simulink model "FCSMPC_double_vector_2025b"  (R2025b)
settings: Solver=FixedStepDiscrete  StartTime=0.0  StopTime=2  FixedStep=SimulinkTs  RelTol=1e-3
PreLoadFcn:
  | % Verzeichnis des Modells zum MATLAB-Pfad hinzufügen
  | modelDir = fileparts(get_param(bdroot, 'FileName'));
  | addpath(modelDir);
  | 
  | % Nur der Dateiname – kein Pfad!
  | set_param(bdroot, 'DataDictionary', 'FOC_params.sldd');
model workspace (MAT data in the model file):
  Np : Simulink.Parameter (value not decoded)
values from neighbouring files (symbols this model uses):
  Filter_Current_FilterTimeConst = 3.3333333333333335E-5    [FOC_params.sldd]
  Filter_Current_SensorTimeConst = 1.5915494309189535E-6    [FOC_params.sldd]
  FOC = evalin("base", "FOC")    [createFOC_SLDD.m]
  FOC_Control_Current_KIid = 10.0    [FOC_params.sldd]
  FOC_Control_Current_KIiq = 10.0    [FOC_params.sldd]
  FOC_Control_Current_KPid = 0.20418507462686566    [FOC_params.sldd]
  FOC_Control_Current_KPiq = 0.58674626865671642    [FOC_params.sldd]
  FOC_Control_Current_Krd = 0.8    [FOC_params.sldd]
  FOC_Control_Current_Krq = 0.8    [FOC_params.sldd]
  FOC_Control_Current_TclCur = 0.1    [FOC_params.sldd]
  FOC_Control_Current_Tnd = 0.1    [FOC_params.sldd]
  FOC_Control_Current_Tnq = 0.1    [FOC_params.sldd]
  FOC_Control_InverterVdc_V = 400.0    [FOC_params.sldd]
  FOC_Control_MotorImax_A = 650.0    [FOC_params.sldd]
  FOC_Control_MTPA_MTPV_nT_id_grid = -450.06704889786266 -439.56177000270145 -427.77784873303676 -416.66404703197372 -406.07553272717422 -395.15516533678584 -384.31176061747851 -374.03652088128132 -363.90551910193739 -353.79478643334204 -344.0221683092833 -334.51243453441936 -324.94614350292119 -315.21793409137081 -305.26543360965195 -295.21828280911944 -285.133916324101 -275.01232812136521 -264.86951532374729 -254.7797625148454 -244    [FOC_params.sldd]
  FOC_Control_MTPA_MTPV_nT_iq_grid = -449.09165648258488 -442.56958748923387 -437.25247759546528 -430.91792082419158 -423.83735797306491 -417.11730433547 -410.54064621830616 -403.71584331167304 -396.93611069310379 -390.15794305727007 -382.97216593027133 -375.44639668848538 -367.93447385667577 -360.57088856352266 -353.41289778449368 -346.34020584402072 -339.28416684923008 -332.22010880540631 -325.11927997033376 -317.92299905654966 -31    [FOC_params.sldd]
  FOC_Control_MTPA_MTPV_T_vec = -245.0 -240.0 -235.0 -230.0 -225.0 -220.0 -215.0 -210.0 -205.0 -200.0 -195.0 -190.0 -185.0 -180.0 -175.0 -170.0 -165.0 -160.0 -155.0 -150.0 -145.0 -140.0 -135.0 -130.0 -125.0 -120.0 -115.0 -110.0 -105.0 -100.0 -95.0 -90.0 -85.0 -80.0 -75.0 -70.0 -65.0 -60.0 -55.0 -50.0 -45.0 -40.0 -35.0 -30.0 -25.0 -20.0 -15.0 -10.0 -5.0 0.0 5.0 10.0 15.0 20.0 25.0 30.0 35.0 40.0 45.0 50.0 55.0 60.0 65.0 70.0 75.0    [FOC_params.sldd]
  FOC_Control_MTPA_MTPV_w_vec = 0.0 10.471975511965978 20.943951023931955 31.415926535897931 41.887902047863911 52.359877559829883 62.831853071795862 73.303828583761828 83.775804095727821 94.247779607693786 104.71975511965977 115.19173063162575 125.66370614359172 136.1356816555577 146.60765716752366 157.07963267948966 167.55160819145564 178.02358370342159 188.49555921538757 198.96753472735358 209.43951023931953 219.9114857512855    [FOC_params.sldd]
  FOC_Control_OpenLoop_Id_Ref_A = 0.0    [FOC_params.sldd]
  FOC_Control_OpenLoop_Iq_Ref_A = 0.0    [FOC_params.sldd]
  FOC_Control_OpenLoop_Ud_OpenLoop_V = 0.0    [FOC_params.sldd]
  FOC_Control_OpenLoop_Uq_OpenLoop_V = 0.0    [FOC_params.sldd]
  FOC_Control_RF_omegamech_rad_s = 3141.5926535897934    [FOC_params.sldd]
  FOC_Control_RF_RateCurrent_A = 500.0    [FOC_params.sldd]
  FOC_Control_RF_RateTrq_Nm = 500.0    [FOC_params.sldd]
  FOC_Control_theta_mechOffsetFix = 0.0    [FOC_params.sldd]
  FOC_Control_theta_mechOffsetTime = 0.0    [FOC_params.sldd]
  FOC_Control_TorqueRef_Nm = 10.0    [FOC_params.sldd]
  FOC_Control_Umax_V = 230.94010767585033    [FOC_params.sldd]
  FOC_Flag_ClosedLoopControl = 1.0    [FOC_params.sldd]
  FOC_Flag_ControlStrategy = 2.0    [FOC_params.sldd]
  FOC_Flag_PWMEnable = 1.0    [FOC_params.sldd]
  FOC_Flag_ResetControl = 0.0    [FOC_params.sldd]
  FOC_Flag_TorqueControl = 1.0    [FOC_params.sldd]
  FOC_LUT_DQLimiter_DQ_LUTScaling = 1.8749999999999995E-5    [FOC_params.sldd]
  FOC_PWM_AZSPWMMethod = 3.0    [FOC_params.sldd]
  FOC_PWM_HybridMode = 1.0    [FOC_params.sldd]
  FOC_PWM_LB1 = 0.5    [FOC_params.sldd]
  FOC_PWM_LB2 = 0.77    [FOC_params.sldd]
  FOC_PWM_PWMManuel = 1.0    [FOC_params.sldd]
  FOC_PWM_RSPWMMethod = 2.0    [FOC_params.sldd]
  FOC_PWM_UB1 = 0.66    [FOC_params.sldd]
  FOC_PWM_UB2 = 0.9    [FOC_params.sldd]
  FOC_SampleTime_TsCur = 0.0001    [FOC_params.sldd]
undefined symbols (not defined in the file or in its folder): dspblkCoreblockFVToolHelper, FCS, Filter, gcbh, Plant, SimulinkTs
libraries: hdlsllib x2, simulink x2, autolibfluxpmsm x1
(part 5 of 8)

== matlab function FCSMPC_double_vector_2025b/FCS_MPC/SDA_Solve/SDA Solve/QP_Runtime_40k_Simplified ==
  data: H input double size=[15 15]; U_unc output double size=[15 1]; Gamma input double size=[10 2]; Phi input double size=[10 1]; Lambdafsw_SE input double size=[15 3]; Upsil input double size=[10 15]; Bd input double size=[2 2]; Bs_TI input double size=[2 3]; deltaIdqBaseOffset input double size=[2 1]; deltaIdqState input double size=[2 2]; magnitudeGain input double size=[1 1]; phaseCompensation input double size=[2 2]; rippleAttenuation input double size=[1 1]; rippleDelay input double size=[1 1]; Sin_Cos_Theta input double size=[2 1]; idiqFiltered input double size=[2 1]; idiq_ref input double size=[2 1]; Ts input double size=[1 1]; U_applied input double size=[6 1]; controllerDelay input double size=[1 1]; iabcPredictedPrevious input double size=[3 1]; Iabc_Motor input double size=[3 1]; predictionValid input boolean size=[1 1]; iabcReconstruction output double size=[3 1]; deltaIabcBase output double size=[3 1]; deltaIabcSwitch output double size=[3 3]; predictionError output double size=[3 1]; reconstructionError output double size=[3 1]; predictionError_dq output double size=[2 1]; reconstructionError_dq output double size=[2 1]; iabcAverageEstimated output double size=[3 1]; iabcRippleEstimated output double size=[3 1]; rippleResidual output double size=[3 1]; iabcSwitchCorrectionRaw output double size=[3 1]
function [U_unc,iabcReconstruction, ...
    deltaIabcBase,deltaIabcSwitch, ...
    predictionError,reconstructionError, ...
    predictionError_dq,reconstructionError_dq, ...
    iabcAverageEstimated,iabcRippleEstimated,rippleResidual, ...
    iabcSwitchCorrectionRaw] = ...
    QP_Runtime_40k_Simplified( ...
    H,Gamma,Phi,Lambdafsw_SE,Upsil,Bd,Bs_TI, ...
    deltaIdqBaseOffset,deltaIdqState, ...
    magnitudeGain,phaseCompensation,rippleAttenuation,rippleDelay, ...
    Sin_Cos_Theta,idiqFiltered,idiq_ref,Ts,U_applied,controllerDelay, ...
    iabcPredictedPrevious,Iabc_Motor,predictionValid)
%#codegen
% Fast-rate current reconstruction, diagnostics, and QP linear solve.
% H/Upsil remain frozen at the 10-kHz midpoint angle. The instantaneous
% current transforms and switching-current increment use the current
% 40-kHz electrical angle so their error does not scale with load current.

Ts = max(realmin('double'),double(Ts));
idiqFiltered = double(idiqFiltered);
idiq_ref = double(idiq_ref);
U_applied = double(U_applied);
Bd = double(Bd);
Bs_TI = double(Bs_TI);
Sin_Cos_Theta = double(Sin_Cos_Theta);
iabcPredictedPrevious = double(iabcPredictedPrevious);
Iabc_Motor = double(Iabc_Motor);
predictionValid = logical(predictionValid);
uFirst = U_applied(1:3);
uSecond = U_applied(4:6);
uAverage = 0.5*(uFirst+uSecond);

sinTheta = Sin_Cos_Theta(1);
cosTheta = Sin_Cos_Theta(2);
Rp = [cosTheta, sinTheta; -sinTheta, cosTheta];
TinvClarke = [1.0, 0.0; ...
             -0.5, sqrt(3)/2; ...
             -0.5, -sqrt(3)/2];
Tclarke = [2/3, -1/3, -1/3; ...
           0, 1/sqrt(3), -1/sqrt(3)];
Tdq2abc = TinvClarke*Rp.';
Tabc2dq = Rp*Tclarke;
deltaIdqSwitch = Bd*Rp*Bs_TI;

% One frozen current-increment model, linearized at idiqFiltered.
deltaIdqBase = deltaIdqState*idiqFiltered+deltaIdqBaseOffset;
period = 2.0*Ts;
rippleAtMeasurementDq = ripple_at_phase( ...
    deltaIdqSwitch,uFirst,uSecond,uAverage, ...
    Ts,period-rippleDelay);
rippleResidualDq = ...
    magnitudeGain*rippleAttenuation*rippleAtMeasurementDq;
idiqAverage = phaseCompensation*( ...
    magnitudeGain*idiqFiltered-rippleResidualDq);
idiqAverage = idiqAverage+(rippleDelay/Ts)*( ...
    deltaIdqBase+deltaIdqSwitch*uAverage);

rippleNow = ripple_at_phase( ...
    deltaIdqSwitch,uFirst,uSecond,uAverage,Ts,period);
idiqAtSample = idiqAverage+rippleNow;
delayRatio = min(max(0.0,double(controllerDelay)),Ts)/Ts;
idiqCompensated = idiqAtSample+delayRatio*( ...
    deltaIdqBase+deltaIdqSwitch*uSecond);

% The only dq-to-abc conversion point in the runtime data path.
iabcReconstruction = Tdq2abc*idiqCompensated;
deltaIabcBase = Tdq2abc*deltaIdqBase;
deltaIabcSwitch = Tdq2abc*deltaIdqSwitch;

% Diagnostic ports match Current_Reconstruction_Switch_Frequency_kHz_Simplified.
iabcAverageEstimated = Tdq2abc*idiqAverage;
iabcRippleEstimated = Tdq2abc*rippleNow;
rippleResidual = Tdq2abc*rippleResidualDq;
iabcAmpCorrected = Tdq2abc*(magnitudeGain*idiqFiltered);
iabcSwitchCorrectionRaw = ...
    (iabcAverageEstimated-iabcAmpCorrected)+iabcRippleEstimated;
if predictionValid
    predictionError = iabcReconstruction-iabcPredictedPrevious;
else
    predictionError = zeros(3,1);
end
reconstructionError = Iabc_Motor-iabcReconstruction;
predictionError_dq = Tabc2dq*predictionError;
reconstructionError_dq = Tabc2dq*reconstructionError;

Np = 5;
r = Gamma*idiqCompensated+Phi-repmat(idiq_ref,Np,1);
F = Upsil.'*r-Lambdafsw_SE*uSecond;
y = H.'\(-F);
U_unc = H\y;
end

function rippleCurrent = ripple_at_phase( ...
    deltaSwitch,uFirst,uSecond,uAverage,vectorStep,t)
period = 2.0*vectorStep;
deltaFirst = deltaSwitch*(uFirst-uAverage);
deltaSecond = deltaSwitch*(uSecond-uAverage);
rippleStart = -0.5*deltaFirst;
t = min(max(0.0,t),period);
if t <= vectorStep
    rippleCurrent = rippleStart+(t/vectorStep)*deltaFirst;
else
    rippleCurrent = rippleStart+deltaFirst+ ...
        ((t-vectorStep)/vectorStep)*deltaSecond;
end
end

== matlab function FCSMPC_double_vector_2025b/FCS_MPC/SDA_Solve/SDA Solve/original ==
  data: Ad input size=[2 2]; iabcReconstruction output size=[3 1]; Bd input size=[2 2]; fd input size=[2 1]; Bs_TI input size=[2 3]; idiqFiltered input size=[2 1]; Sin_Cos_Theta input size=[2 1]; wel input; Ts input; U_applied input size=[6 1]; controllerDelay input; iabcPredictedPrevious input size=[3 1]; Iabc_Motor input; predictionValid input; filterTimeConstant input; sensorTimeConstant input; filterDelayGain input; idiqCompensated output size=[2 1]; deltaIabcBase output size=[3 1]; deltaIabcSwitch output size=[3 3]; Bs output size=[2 3]; predictionError output size=[3 1]; reconstructionError output size=[3 1]; predictionError_dq output; reconstructionError_dq output; iabcAverageEstimated output size=[3 1]; iabcRippleEstimated output size=[3 1]; rippleResidual output; iabcSwitchCorrectionRaw output
function [iabcReconstruction,idiqCompensated, ...
    deltaIabcBase,deltaIabcSwitch,Bs, ...
    predictionError,reconstructionError, ...
    predictionError_dq,reconstructionError_dq, ...
    iabcAverageEstimated,iabcRippleEstimated,rippleResidual,...
    iabcSwitchCorrectionRaw] = ...
    Current_Reconstruction_Switch_Frequency_kHz( ...
    Ad,Bd,fd,Bs_TI,idiqFiltered, ...
    Sin_Cos_Theta,wel,Ts,U_applied,controllerDelay, ...
    iabcPredictedPrevious,Iabc_Motor,predictionValid, ...
    filterTimeConstant,sensorTimeConstant,filterDelayGain)
% Input dimensions:
%   Ad, Bd                    2x2
%   fd                        2x1
%   Bs_TI                     2x3
%   idiqFiltered              2x1
%   Sin_Cos_Theta             2x1 = [sin(theta); cos(theta)]
%   U_applied                 6x1 = [uFirst; uSecond]
%   iabcPredictedPrevious     3x1
%   Iabc_Motor                3x1 (simulation/reference measurement only)
%   all remaining inputs      scalar
%
% Output dimensions:
%   iabcReconstruction        3x1
%   idiqCompensated           2x1
%   deltaIabcBase             3x1
%   deltaIabcSwitch           3x3
%   Bs                        2x3
%   predictionError           3x1 = reconstruction - previous prediction
%   reconstructionError       3x1 = motor current - reconstruction
%   predictionError_dq        2x1
%   reconstructionError_dq    2x1
%   iabcAverageEstimated      3x1
%   iabcRippleEstimated       3x1
%   iabcSwitchCorrectionRaw   3x1

Ad = double(Ad);
Bd = double(Bd);
fd = double(fd);
Bs_TI = double(Bs_TI);
idiqFiltered = double(idiqFiltered);
Sin_Cos_Theta = double(Sin_Cos_Theta);
wel = double(wel);
Ts = max(realmin('double'),double(Ts));
% Ts is one SDA vector step and equals 0.5*MPC_Ts in the Simulink model.
% The complete double-vector ripple period is 2*Ts.
vectorStep = Ts;
doubleVectorPeriod = 2.0*vectorStep;
U_applied = double(U_applied);
controllerDelay = max(0.0,double(controllerDelay));
iabcPredictedPrevious = double(iabcPredictedPrevious);
Iabc_Motor = double(Iabc_Motor);
predictionValid = logical(predictionValid);
filterTimeConstant = max(0.0,double(filterTimeConstant));
sensorTimeConstant = max(0.0,double(sensorTimeConstant));
filterDelayGain = max(0.0,double(filterDelayGain));

sinTheta = Sin_Cos_Theta(1);
cosTheta = Sin_Cos_Theta(2);
Tc = [2/3, -1/3, -1/3; ...
       0, 1/sqrt(3), -1/sqrt(3)];
Rp = [cosTheta, sinTheta; -sinTheta, cosTheta];
TinvClarke = [1.0, 0.0; ...
      -0.5, sqrt(3)/2; ...
      -0.5, -sqrt(3)/2];
Tdq2abc = TinvClarke*Rp.';

uFirst = U_applied(1:3);
uSecond = U_applied(4:6);
uAverage = 0.5*(uFirst+uSecond);

% Fundamental inverse-filter magnitude and phase at electrical frequency.
omegaFilter = wel*filterTimeConstant;
omegaSensor = wel*sensorTimeConstant;
magnitudeGain = sqrt(1.0+omegaFilter*omegaFilter)*sqrt(1.0+omegaSensor*omegaSensor);
iabcAmpCorrected = magnitudeGain*(Tdq2abc*idiqFiltered);

% basePhaseDelay belongs to the fundamental component. The empirical
% rippleReconstructionDelay is scheduled from it but is used only to locate
% the switching ripple contained in the filtered measurement.
w = abs(wel);
if w > 1.0e-6
    basePhaseDelay = (atan(w*filterTimeConstant)+ ...
        atan(w*sensorTimeConstant))/w;
else
    basePhaseDelay = filterTimeConstant+sensorTimeConstant;
end

% The filtered measurement still contains an attenuated switching ripple
% from the delayed phase. Remove that residual before treating the signal as
% the filtered base current. Because iabcAmpCorrected has already been
% scaled by magnitudeGain, apply the same scale to the residual ripple.
[~,deltaSwitchAtSample,~,~] = abc_current_increment( ...
    iabcAmpCorrected,Ad,Bd,fd,Bs_TI,wel,Ts,Tc,Rp,Tdq2abc);
% Fixed carrier-frequency comparison. Express the frequency in kHz for
% direct tuning and convert it to angular frequency only once here.
% This replaces omegaSwitch = 2*pi/doubleVectorPeriod; all other equations
% are identical to Current_Reconstruction_Switch_Frequency.
switchFrequency_kHz = 17.0;
omegaSwitch = 2.0*pi*switchFrequency_kHz*1.0e3;
omegaRipple = max(1.0,omegaSwitch);
omegaRippleFilter = omegaRipple*filterTimeConstant;
omegaRippleSensor = omegaRipple*sensorTimeConstant;
rippleAttenuation = 1.0/( ...
    sqrt(1.0+omegaRippleFilter*omegaRippleFilter)* ...
    sqrt(1.0+omegaRippleSensor*omegaRippleSensor));
rippleReconstructionDelay = ...
    (atan(omegaRipple*filterTimeConstant)+ ...
    atan(omegaRipple*sensorTimeConstant))/omegaRipple;
rippleReconstructionDelay = min(max(0.0,rippleReconstructionDelay),doubleVectorPeriod);
samplePhase = doubleVectorPeriod;
rippleMeasurementPhase = samplePhase-rippleReconstructionDelay;
rippleAtMeasurement = double_vector_ripple_at_phase( ...
    deltaSwitchAtSample,uFirst,uSecond,uAverage,vectorStep, ...
    rippleMeasurementPhase);

% Residual switching ripple remaining in the amplitude-corrected measurement.
rippleResidual = magnitudeGain*rippleAttenuation*rippleAtMeasurement;

% Fundamental with correct magnitude but still carrying the filter phase lag.
iabcBaseLagged = iabcAmpCorrected-rippleResidual;

% Explicit fundamental phase compensation. Rotate the stationary
% alpha-beta current vector by the signed filter phase error.
phaseCompensation = wel*basePhaseDelay;
cosPhaseComp = cos(phaseCompensation);
sinPhaseComp = sin(phaseCompensation);
phaseCompMatrix = [cosPhaseComp, -sinPhaseComp; ...
                   sinPhaseComp,  cosPhaseComp];
iabBeforePhaseComp = Tc*iabcBaseLagged;
iabAfterPhaseComp = phaseCompMatrix*iabBeforePhaseComp;
iabcAverageEstimated = TinvClarke*iabAfterPhaseComp;

% Restore the average current evolution over the ripple reconstruction
% interval. This is the state-space increment produced by the motor dynamics
% and the average of the two actually applied switching states; it is kept
% separate from the fundamental inverse-filter phase correction above.
if rippleReconstructionDelay > 0.0
    [deltaBase,deltaSwitch,~,~] = abc_current_increment( ...
        iabcAverageEstimated,Ad,Bd,fd,Bs_TI,wel,Ts,Tc,Rp,Tdq2abc);
    averageCurrentIncrement = (rippleReconstructionDelay/Ts)*( ...
        deltaBase+deltaSwitch*uAverage);
    iabcAverageEstimated = ...
        iabcAverageEstimated+averageCurrentIncrement;
end

% Re-evaluate the sensitivity at the reconstructed average and restore the
% piecewise triangular ripple at the present sampling boundary.
[~,deltaSwitchAtSample,~,~] = abc_current_increment( ...
    iabcAverageEstimated,Ad,Bd,fd,Bs_TI,wel,Ts,Tc,Rp,Tdq2abc);
iabcRippleEstimated = double_vector_ripple_at_phase( ...
    deltaSwitchAtSample,uFirst,uSecond,uAverage,vectorStep,samplePhase);

% Raw diagnostic correction relative to the magnitude-corrected measurement.
iabcSwitchCorrectionRaw = ...
    (iabcAverageEstimated-iabcAmpCorrected)+iabcRippleEstimated;
iabcAtSample = iabcAverageEstimated+iabcRippleEstimated;

% External controller delay is separate from the filter delay. The final
% applied vector remains active until the new command becomes effective.
effectiveControllerDelay = min(controllerDelay,Ts);
[deltaBase,deltaSwitch,~,~] = abc_current_increment( ...
    iabcAtSample,Ad,Bd,fd,Bs_TI,wel,Ts,Tc,Rp,Tdq2abc);
iabcReconstruction = iabcAtSample+(effectiveControllerDelay/Ts)*( ...
    deltaBase+deltaSwitch*uSecond);

[deltaIabcBase,deltaIabcSwitch,idiqCompensated,Bs] = ...
    abc_current_increment(iabcReconstruction,Ad,Bd,fd,Bs_TI,wel,Ts, ...
    Tc,Rp,Tdq2abc);

if predictionValid
    predictionError = iabcReconstruction-iabcPredictedPrevious;
else
    predictionError = zeros(3,1);
end
reconstructionError = Iabc_Motor-iabcReconstruction;
predictionError_dq = Rp*(Tc*predictionError);
reconstructionError_dq = Rp*(Tc*reconstructionError);
end

function [deltaBase,deltaSwitch,idiqState,Bs] = abc_current_increment( ...
    iabc,Ad,Bd,fd,Bs_TI,wel,Ts,Tc,Rp,Tdq2abc)
% One-vector-step PMSM current increment. Ts = 0.5*MPC_Ts, and Ad/Bd/fd
% are discretized using this same vector-step duration.
Jrot = [0 -1; 1 0];
idiqState = Rp*(Tc*iabc);
Bs = Bd*Rp*Bs_TI;
deltaIdqBase = (Ad-eye(2))*idiqState+fd;
deltaBase = Tdq2abc*(deltaIdqBase+Jrot*idiqState*(wel*Ts));
deltaSwitch = Tdq2abc*Bs;
end

function rippleCurrent = double_vector_ripple_at_phase( ...
    deltaSwitchAtSample,uFirst,uSecond,uAverage,vectorStep,t)
doubleVectorPeriod = 2.0*vectorStep;
deltaFirstVectorStep = ...
    deltaSwitchAtSample*(uFirst-uAverage);
deltaSecondVectorStep = ...
    deltaSwitchAtSample*(uSecond-uAverage);
rippleAtPeriodStart = -0.5*deltaFirstVectorStep;
t = min(max(0.0,t),doubleVectorPeriod);
if t <= vectorStep
    rippleCurrent = rippleAtPeriodStart+ ...
        (t/vectorStep)*deltaFirstVectorStep;
else
    rippleCurrent = rippleAtPeriodStart+deltaFirstVectorStep+ ...
        ((t-vectorStep)/vectorStep)*deltaSecondVectorStep;
end
end

== matlab function FCSMPC_double_vector_2025b/FCS_MPC/SDA_Solve/SDA Solve/simplified ==
  data: Ad input size=[2 2]; iabcReconstruction output size=[3 1]; Bd input size=[2 2]; fd input size=[2 1]; Bs_TI input size=[2 3]; idiqFiltered input size=[2 1]; Sin_Cos_Theta input size=[2 1]; wel input size=1; Ts input size=1; U_applied input size=[6 1]; controllerDelay input size=1; iabcPredictedPrevious input size=[3 1]; Iabc_Motor input size=[3 1]; predictionValid input; filterTimeConstant input; sensorTimeConstant input; filterDelayGain input; idiqCompensated output size=[2 1]; deltaIabcBase output size=[3 1]; deltaIabcSwitch output size=[3 3]; Bs output size=[2 3]; predictionError output size=[3 1]; reconstructionError output size=[3 1]; predictionError_dq output; reconstructionError_dq output; iabcAverageEstimated output size=[3 1]; iabcRippleEstimated output size=[3 1]; rippleResidual output; iabcSwitchCorrectionRaw output
function [iabcReconstruction,idiqCompensated, ...
    deltaIabcBase,deltaIabcSwitch,Bs, ...
    predictionError,reconstructionError, ...
    predictionError_dq,reconstructionError_dq, ...
    iabcAverageEstimated,iabcRippleEstimated,rippleResidual, ...
    iabcSwitchCorrectionRaw] = ...
    Current_Reconstruction_Switch_Frequency_kHz_Simplified( ...
    Ad,Bd,fd,Bs_TI,idiqFiltered,Sin_Cos_Theta,wel,Ts,U_applied, ...
    controllerDelay,iabcPredictedPrevious,Iabc_Motor,predictionValid, ...
    filterTimeConstant,sensorTimeConstant,filterDelayGain)
%#codegen
% Simplified reconstruction using one current-increment linearization.
% All internal current calculations remain in dq.  idiqFiltered is used as
% the single linearization state; conversion to abc occurs only for outputs.
% The interface intentionally matches Current_Reconstruction_Switch_Frequency_kHz
% so the two implementations can be exchanged directly for error evaluation.

Ad = double(Ad);
Bd = double(Bd);
fd = double(fd);
Bs_TI = double(Bs_TI);
idiqFiltered = double(idiqFiltered);
Sin_Cos_Theta = double(Sin_Cos_Theta);
wel = double(wel);
Ts = max(realmin('double'),double(Ts));
U_applied = double(U_applied);
controllerDelay = max(0.0,double(controllerDelay));
iabcPredictedPrevious = double(iabcPredictedPrevious);
Iabc_Motor = double(Iabc_Motor);
predictionValid = logical(predictionValid);
filterTimeConstant = max(0.0,double(filterTimeConstant));
sensorTimeConstant = max(0.0,double(sensorTimeConstant));
filterDelayGain = double(filterDelayGain); %#ok<NASGU> retained for interface compatibility

sinTheta = Sin_Cos_Theta(1);
cosTheta = Sin_Cos_Theta(2);
Rp = [cosTheta, sinTheta; -sinTheta, cosTheta];
TinvClarke = [1.0, 0.0; ...
             -0.5, sqrt(3)/2; ...
             -0.5, -sqrt(3)/2];
Tdq2abc = TinvClarke*Rp.';

uFirst = U_applied(1:3);
uSecond = U_applied(4:6);
uAverage = 0.5*(uFirst+uSecond);

% The only current-increment evaluation.  Later propagation deliberately
% reuses this local model instead of repeatedly re-linearizing reconstructed
% abc currents and transforming them back to dq.
Jrot = [0 -1; 1 0];
BsDq = Bd*Rp*Bs_TI;
Bs = BsDq;
deltaIdqBase = (Ad-eye(2))*idiqFiltered+fd+ ...
    Jrot*idiqFiltered*(wel*Ts);
deltaIdqSwitch = BsDq;

omegaFilter = wel*filterTimeConstant;
omegaSensor = wel*sensorTimeConstant;
magnitudeGain = sqrt(1.0+omegaFilter*omegaFilter)* ...
    sqrt(1.0+omegaSensor*omegaSensor);

w = abs(wel);
if w > 1.0e-6
    basePhaseDelay = (atan(w*filterTimeConstant)+ ...
        atan(w*sensorTimeConstant))/w;
else
    basePhaseDelay = filterTimeConstant+sensorTimeConstant;
end

vectorStep = Ts;
doubleVectorPeriod = 2.0*vectorStep;
omegaRipple = 2.0*pi*17.0e3;
omegaRippleFilter = omegaRipple*filterTimeConstant;
omegaRippleSensor = omegaRipple*sensorTimeConstant;
rippleAttenuation = 1.0/( ...
    sqrt(1.0+omegaRippleFilter*omegaRippleFilter)* ...
    sqrt(1.0+omegaRippleSensor*omegaRippleSensor));
rippleDelay = (atan(omegaRipple*filterTimeConstant)+ ...
    atan(omegaRipple*sensorTimeConstant))/omegaRipple;
rippleDelay = min(max(0.0,rippleDelay),doubleVectorPeriod);

rippleAtMeasurementDq = double_vector_ripple_at_phase( ...
    deltaIdqSwitch,uFirst,uSecond,uAverage,vectorStep, ...
    doubleVectorPeriod-rippleDelay);
rippleResidualDq = magnitudeGain*rippleAttenuation*rippleAtMeasurementDq;

phase = wel*basePhaseDelay;
phaseCompensation = [cos(phase), -sin(phase); ...
                     sin(phase),  cos(phase)];
idiqAverageEstimated = phaseCompensation*( ...
    magnitudeGain*idiqFiltered-rippleResidualDq);

% Reuse the increment frozen at idiqFiltered, as requested.
idiqAverageEstimated = idiqAverageEstimated+(rippleDelay/Ts)*( ...
    deltaIdqBase+deltaIdqSwitch*uAverage);
rippleAtSampleDq = double_vector_ripple_at_phase( ...
    deltaIdqSwitch,uFirst,uSecond,uAverage,vectorStep,doubleVectorPeriod);
idiqAtSample = idiqAverageEstimated+rippleAtSampleDq;

delayRatio = min(controllerDelay,Ts)/Ts;
idiqCompensated = idiqAtSample+delayRatio*( ...
    deltaIdqBase+deltaIdqSwitch*uSecond);

% Convert to abc once, at the output boundary.
iabcReconstruction = Tdq2abc*idiqCompensated;
deltaIabcBase = Tdq2abc*deltaIdqBase;
deltaIabcSwitch = Tdq2abc*deltaIdqSwitch;
iabcAverageEstimated = Tdq2abc*idiqAverageEstimated;
iabcRippleEstimated = Tdq2abc*rippleAtSampleDq;
rippleResidual = Tdq2abc*rippleResidualDq;

% Diagnostics are evaluated only after the final dq-domain reconstruction.
% They therefore preserve the original interface without introducing extra
% abc-to-dq round trips into the reconstruction algorithm itself.
iabcAmpCorrected = Tdq2abc*(magnitudeGain*idiqFiltered);
iabcSwitchCorrectionRaw = ...
    (iabcAverageEstimated-iabcAmpCorrected)+iabcRippleEstimated;
if predictionValid
    predictionError = iabcReconstruction-iabcPredictedPrevious;
else
    predictionError = zeros(3,1);
end
reconstructionError = Iabc_Motor-iabcReconstruction;
predictionError_dq = Rp*clarke_transform(predictionError);
reconstructionError_dq = Rp*clarke_transform(reconstructionError);
end

function iab = clarke_transform(iabc)
iab = [2/3, -1/3, -1/3; ...
       0, 1/sqrt(3), -1/sqrt(3)]*iabc;
end

function rippleCurrent = double_vector_ripple_at_phase( ...
    deltaSwitch,uFirst,uSecond,uAverage,vectorStep,t)
period = 2.0*vectorStep;
deltaFirst = deltaSwitch*(uFirst-uAverage);
deltaSecond = deltaSwitch*(uSecond-uAverage);
rippleStart = -0.5*deltaFirst;
t = min(max(0.0,t),period);
if t <= vectorStep
    rippleCurrent = rippleStart+(t/vectorStep)*deltaFirst;
else
    rippleCurrent = rippleStart+deltaFirst+ ...
        ((t-vectorStep)/vectorStep)*deltaSecond;
end
end

== matlab function FCSMPC_double_vector_2025b/FCS_MPC/SDA_Solve/SDA Solve/QP_Runtime_40k_Simplified_embedded_H ==
  data: H input double size=[15 15]; U_unc output double size=[15 1]; Gamma input double size=[10 2]; Phi input double size=[10 1]; Lambdafsw_SE input double size=[15 3]; Upsil input double size=[10 15]; Bd input double size=[2 2]; Bs_TI input double size=[2 3]; deltaIdqBaseOffset input double size=[2 1]; deltaIdqState input double size=[2 2]; magnitudeGain input double size=[1 1]; phaseCompensation input double size=[2 2]; rippleAttenuation input double size=[1 1]; rippleDelay input double size=[1 1]; Sin_Cos_Theta input double size=[2 1]; idiqFiltered input double size=[2 1]; idiq_ref input double size=[2 1]; lambdaZeroEmbedded input; Ts input double size=[1 1]; U_applied input double size=[6 1]; controllerDelay input double size=[1 1]; iabcPredictedPrevious input double size=[3 1]; Iabc_Motor input double size=[3 1]; predictionValid input boolean size=[1 1]; iabcReconstruction output double size=[3 1]; deltaIabcBase output double size=[3 1]; deltaIabcSwitch output double size=[3 3]; predictionError output double size=[3 1]; reconstructionError output double size=[3 1]; predictionError_dq output double size=[2 1]; reconstructionError_dq output double size=[2 1]; iabcAverageEstimated output double size=[3 1]; iabcRippleEstimated output double size=[3 1]; rippleResidual output double size=[3 1]; iabcSwitchCorrectionRaw output double size=[3 1]
function [U_unc,iabcReconstruction, ...
    deltaIabcBase,deltaIabcSwitch, ...
    predictionError,reconstructionError, ...
    predictionError_dq,reconstructionError_dq, ...
    iabcAverageEstimated,iabcRippleEstimated,rippleResidual, ...
    iabcSwitchCorrectionRaw] = ...
    QP_Runtime_40k_Simplified_ZeroVectorEmbedded( ...
    H,Gamma,Phi,Lambdafsw_SE,Upsil,Bd,Bs_TI, ...
    deltaIdqBaseOffset,deltaIdqState, magnitudeGain,phaseCompensation,...
    rippleAttenuation,rippleDelay,Sin_Cos_Theta,idiqFiltered, ...
    idiq_ref,lambdaZeroEmbedded,Ts,U_applied,controllerDelay, ...
    iabcPredictedPrevious,Iabc_Motor,predictionValid)
%#codegen
% Fast-rate reconstruction and QP solve for the embedded-zero-vector model.
% H already contains the quadratic zero-vector term. Its matching linear
% term is rebuilt locally from the scalar lambdaZeroEmbedded, avoiding a
% 15-element data transfer from the 10-kHz precomputation. The additive
% constant is irrelevant.
% The separate commanded-zero-vector penalty in SDA must be set to zero to
% prevent double counting. A distinct dead-time CMV penalty may remain.

Ts = max(realmin('double'),double(Ts));
idiqFiltered = double(idiqFiltered);
idiq_ref = double(idiq_ref);
U_applied = double(U_applied);
lambdaZeroEmbedded = max(0.0,double(lambdaZeroEmbedded));
Bd = double(Bd);
Bs_TI = double(Bs_TI);
Sin_Cos_Theta = double(Sin_Cos_Theta);
iabcPredictedPrevious = double(iabcPredictedPrevious);
Iabc_Motor = double(Iabc_Motor);
predictionValid = logical(predictionValid);
uFirst = U_applied(1:3);
uSecond = U_applied(4:6);
uAverage = 0.5*(uFirst+uSecond);

sinTheta = Sin_Cos_Theta(1);
cosTheta = Sin_Cos_Theta(2);
Rp = [cosTheta, sinTheta; -sinTheta, cosTheta];
TinvClarke = [1.0, 0.0; ...
             -0.5, sqrt(3)/2; ...
             -0.5, -sqrt(3)/2];
Tclarke = [2/3, -1/3, -1/3; ...
           0, 1/sqrt(3), -1/sqrt(3)];
Tdq2abc = TinvClarke*Rp.';
Tabc2dq = Rp*Tclarke;
deltaIdqSwitch = Bd*Rp*Bs_TI;

% One frozen current-increment model, linearized at idiqFiltered.
deltaIdqBase = deltaIdqState*idiqFiltered+deltaIdqBaseOffset;
period = 2.0*Ts;
rippleAtMeasurementDq = ripple_at_phase( ...
    deltaIdqSwitch,uFirst,uSecond,uAverage, ...
    Ts,period-rippleDelay);
rippleResidualDq = ...
    magnitudeGain*rippleAttenuation*rippleAtMeasurementDq;
idiqAverage = phaseCompensation*( ...
    magnitudeGain*idiqFiltered-rippleResidualDq);
idiqAverage = idiqAverage+(rippleDelay/Ts)*( ...
    deltaIdqBase+deltaIdqSwitch*uAverage);

rippleNow = ripple_at_phase( ...
    deltaIdqSwitch,uFirst,uSecond,uAverage,Ts,period);
idiqAtSample = idiqAverage+rippleNow;
delayRatio = min(max(0.0,double(controllerDelay)),Ts)/Ts;
idiqCompensated = idiqAtSample+delayRatio*( ...
    deltaIdqBase+deltaIdqSwitch*uSecond);

% The only dq-to-abc conversion point in the runtime data path.
iabcReconstruction = Tdq2abc*idiqCompensated;
deltaIabcBase = Tdq2abc*deltaIdqBase;
deltaIabcSwitch = Tdq2abc*deltaIdqSwitch;

% Diagnostic ports match Current_Reconstruction_Switch_Frequency_kHz_Simplified.
iabcAverageEstimated = Tdq2abc*idiqAverage;
iabcRippleEstimated = Tdq2abc*rippleNow;
rippleResidual = Tdq2abc*rippleResidualDq;
iabcAmpCorrected = Tdq2abc*(magnitudeGain*idiqFiltered);
iabcSwitchCorrectionRaw = ...
    (iabcAverageEstimated-iabcAmpCorrected)+iabcRippleEstimated;
if predictionValid
    predictionError = iabcReconstruction-iabcPredictedPrevious;
else
    predictionError = zeros(3,1);
end
reconstructionError = Iabc_Motor-iabcReconstruction;
predictionError_dq = Tabc2dq*predictionError;
reconstructionError_dq = Tabc2dq*reconstructionError;

Np = 5;
r = Gamma*idiqCompensated+Phi-repmat(idiq_ref,Np,1);
FzeroEmbedded = -0.75*lambdaZeroEmbedded*ones(3*Np,1);
F = Upsil.'*r-Lambdafsw_SE*uSecond+FzeroEmbedded;
y = H.'\(-F);
U_unc = H\y;
end

function rippleCurrent = ripple_at_phase( ...
    deltaSwitch,uFirst,uSecond,uAverage,vectorStep,t)
period = 2.0*vectorStep;
deltaFirst = deltaSwitch*(uFirst-uAverage);
deltaSecond = deltaSwitch*(uSecond-uAverage);
rippleStart = -0.5*deltaFirst;
t = min(max(0.0,t),period);
if t <= vectorStep
    rippleCurrent = rippleStart+(t/vectorStep)*deltaFirst;
else
    rippleCurrent = rippleStart+deltaFirst+ ...
        ((t-vectorStep)/vectorStep)*deltaSecond;
end
end

== matlab function FCSMPC_double_vector_2025b/FCS_MPC/BuildModel/BuildModel/QP_Precompute_10k_Simplified_embedded_H ==
  data: Ld input double size=[1 1]; H output double size=[15 15]; Lq input double size=[1 1]; Rs input double size=[1 1]; Psi input double size=[1 1]; wel input double size=[1 1]; Ts input double size=[1 1]; Vdc input double size=[1 1]; lambda_fsw input double size=[1 1]; lambdaZeroEmbedded input; Sin_Cos_Theta input double size=[2 1]; filterTimeConstant input double size=[1 1]; sensorTimeConstant input double size=[1 1]; Gamma output double size=[10 2]; Phi output double size=[10 1]; Lambdafsw_SE output double size=[15 3]; Upsil output double size=[10 15]; Bd output double size=[2 2]; Bs_TI output double size=[2 3]; deltaIdqBaseOffset output double size=[2 1]; deltaIdqState output double size=[2 2]; magnitudeGain output double size=[1 1]; phaseCompensation output double size=[2 2]; rippleAttenuation output double size=[1 1]; rippleDelay output double size=[1 1]
function [H,Gamma,Phi,Lambdafsw_SE,Upsil, ...
    Bd,Bs_TI,deltaIdqBaseOffset,deltaIdqState, ...
    magnitudeGain,phaseCompensation,rippleAttenuation,rippleDelay] = ...
    QP_Precompute_10k_Simplified_ZeroVectorEmbedded( ...
    Ld,Lq,Rs,Psi,wel,Ts,Vdc,lambda_fsw,lambdaZeroEmbedded, ...
    Sin_Cos_Theta,filterTimeConstant,sensorTimeConstant)
%#codegen
% Slow-rate model/QP preparation with an exactly embedded zero-vector cost.
%
% For every three-bit switching vector u_j, let m_j = [1 1 1]*u_j.
% On the binary domain, m_j belongs to {0,1,2,3}, and
%
%   c0(u_j) = 0.5*(m_j-1)*(m_j-2)
%
% is exactly one for 000 and 111 and zero for all active vectors. Hence
%
%   lambdaZeroEmbedded*c0(u_j)
%     = u_j.'*(0.5*lambdaZeroEmbedded*ones(3))*u_j ...
%       + 2*(-0.75*lambdaZeroEmbedded*ones(3,1)).'*u_j ...
%       + lambdaZeroEmbedded.
%
% The quadratic term is embedded in H here. The matching linear term is
% rebuilt directly from the scalar lambdaZeroEmbedded in the 40-kHz
% runtime calculation, so no 15-element coefficient vector is transferred
% between the two rate domains. The constant Np*lambdaZeroEmbedded is
% omitted because it cannot change the minimizer.
% Set the separate zero-vector penalty in SDA to zero when this formulation
% is used; otherwise the commanded zero-vector cost is counted twice.

Np = 5;
nu = 3;
ny = 2;
Ts = max(realmin('double'),double(Ts));
filterTimeConstant = max(0.0,double(filterTimeConstant));
sensorTimeConstant = max(0.0,double(sensorTimeConstant));
lambdaZeroEmbedded = max(0.0,double(lambdaZeroEmbedded));

Ac = [-Rs/Ld, wel*Lq/Ld; -wel*Ld/Lq, -Rs/Lq];
Bc = [1/Ld, 0; 0, 1/Lq];
fc = [0; -wel*Psi/Lq];
M = [Ac, Bc, fc; zeros(3,5)];
Md = expm(M*Ts);
Ad = Md(1:2,1:2);
Bd = Md(1:2,3:4);
fd = Md(1:2,5);

Apow = zeros(ny*(Np+1),ny);
Apow(1:ny,:) = eye(ny);
for m = 1:Np
    Apow(m*ny+(1:ny),:) = Apow((m-1)*ny+(1:ny),:)*Ad;
end

Gamma = zeros(ny*Np,ny);
Phi = zeros(ny*Np,1);
for i = 1:Np
    rows = (i-1)*ny+(1:ny);
    Gamma(rows,:) = Apow(i*ny+(1:ny),:);
    acc = zeros(ny,1);
    for m = 0:i-1
        acc = acc+Apow(m*ny+(1:ny),:)*fd;
    end
    Phi(rows) = acc;
end

S = eye(nu*Np);
for i = 2:Np
    S((i-1)*nu+(1:nu),(i-2)*nu+(1:nu)) = -eye(nu);
end
E = [eye(nu); zeros(nu*(Np-1),nu)];
lambdaEffective = max(lambda_fsw,1.0e-6);
Lambdafsw_SE = lambdaEffective*(S.'*E);
Lambdafsw_Ssquare = lambdaEffective*(S.'*S);

% Exact quadratic coefficient of the zero-vector indicator.
WzeroEmbedded = 0.5*lambdaZeroEmbedded* ...
    kron(eye(Np),ones(nu));

% One common midpoint electrical angle for the entire controller model.
sinTheta = Sin_Cos_Theta(1);
cosTheta = Sin_Cos_Theta(2);
deltaTheta = wel*50.0e-6;
sinDelta = sin(deltaTheta);
cosDelta = cos(deltaTheta);
sinMid = sinTheta*cosDelta+cosTheta*sinDelta;
cosMid = cosTheta*cosDelta-sinTheta*sinDelta;
RpMid = [cosMid, sinMid; -sinMid, cosMid];
Msw = eye(3)-ones(3)/3;
Tc = (2/3)*[1, -1/2, -1/2; 0, sqrt(3)/2, -sqrt(3)/2];
Bs_TI = Tc*Vdc*Msw;
deltaIdqSwitchMid = Bd*RpMid*Bs_TI;
Jrot = [0 -1; 1 0];
deltaIdqState = Ad-eye(2)+Jrot*(wel*Ts);
deltaIdqBaseOffset = fd;

Upsil = zeros(ny*Np,nu*Np);
for i = 1:Np
    rows = (i-1)*ny+(1:ny);
    for j = 1:i
        cols = (j-1)*nu+(1:nu);
        Upsil(rows,cols) = ...
            Apow((i-j)*ny+(1:ny),:)*deltaIdqSwitchMid;
    end
end

W = Upsil.'*Upsil+Lambdafsw_Ssquare+WzeroEmbedded;
W = 0.5*(W+W.');
W = W+1.0e-12*max(1.0,norm(W,'fro'))*eye(nu*Np);
Jx = fliplr(eye(nu*Np));
[Rt,p] = chol(Jx*W*Jx);
if p ~= 0
    error('H is not positive definite. Increase lambda_sw.');
end
H = Jx*Rt*Jx;

% Angle/frequency-related filter coefficients are also slow-rate values.
omegaFilter = wel*filterTimeConstant;
omegaSensor = wel*sensorTimeConstant;
magnitudeGain = sqrt(1.0+omegaFilter*omegaFilter)* ...
    sqrt(1.0+omegaSensor*omegaSensor);
w = abs(wel);
if w > 1.0e-6
    basePhaseDelay = (atan(w*filterTimeConstant)+ ...
        atan(w*sensorTimeConstant))/w;
else
    basePhaseDelay = filterTimeConstant+sensorTimeConstant;
end
phase = wel*basePhaseDelay;
phaseCompensation = ...
    [cos(phase), -sin(phase); sin(phase), cos(phase)];

omegaRipple = 2.0*pi*17.0e3;
xFilter = omegaRipple*filterTimeConstant;
xSensor = omegaRipple*sensorTimeConstant;
rippleAttenuation = 1.0/(sqrt(1.0+xFilter*xFilter)* ...
    sqrt(1.0+xSensor*xSensor));
rippleDelay = (atan(xFilter)+atan(xSensor))/omegaRipple;
rippleDelay = min(max(0.0,rippleDelay),2.0*Ts);
end

== matlab function FCSMPC_double_vector_2025b/FCS_MPC/SDA_Solve/SDA Solve/PSPL_TestFrame/SDA_PL_Framework/BranchMemory ==
  data: clear input boolean size=[1 1]; initWrite input boolean size=[1 1]; memory output Bus: SdaMemoryBus size=[1 1]; pathWrite input boolean size=[1 1]; vectorWrite input boolean size=[1 1]; level input uint8 size=[1 1]; fsmState input uint8 size=[1 1]; candidate input boolean size=[1 1]; quadraticMetric input double size=[1 1]; vectorMetric input double size=[1 1]; cmvMetric input double size=[1 1]; iabcNext input double size=[3 1]; z input double size=[15 1]; iabcInitial input double size=[3 1]; candidateExhausted output boolean size=[1 1]
function [memory,candidateExhausted] = BranchMemory(clear,initWrite,pathWrite,vectorWrite,level,fsmState,candidate,quadraticMetric,vectorMetric,cmvMetric,iabcNext,z,iabcInitial)
%#codegen
persistent state
if isempty(state)
    state.Uwork=false(15,1);
    state.candidatePosition=ones(15,1,'uint8');
    state.metricStack=zeros(16,1); state.cmvMetricStack=zeros(16,1);
    state.iabcPrediction=zeros(3,6); state.z=zeros(15,1);
end
idx=max(uint8(1),min(uint8(15),level));
if clear
    state.Uwork(:)=false; state.candidatePosition(:)=uint8(1);
    state.metricStack(:)=0.0; state.cmvMetricStack(:)=0.0;
    state.iabcPrediction(:)=0.0; state.z(:)=0.0;
end
if initWrite
    state.z=z; state.iabcPrediction(:,1)=iabcInitial;
    state.metricStack(1)=0.0; state.cmvMetricStack(1)=0.0;
end
if pathWrite
    if fsmState==uint8(7)
        state.Uwork(idx)=candidate;
        state.candidatePosition(idx)=state.candidatePosition(idx)+uint8(1);
        state.metricStack(double(idx)+1)=quadraticMetric;
        state.cmvMetricStack(double(idx)+1)=state.cmvMetricStack(double(idx));
    elseif fsmState==uint8(15)
        state.candidatePosition(idx)=uint8(1);
    elseif fsmState==uint8(17)
        resetIdx=min(uint8(15),idx+uint8(1));
        state.candidatePosition(resetIdx)=uint8(1);
    end
end
if vectorWrite
    state.metricStack(double(idx)+1)=vectorMetric;
    state.cmvMetricStack(double(idx)+1)=cmvMetric;
    predictionStep=idivide(idx,uint8(3));
    currentColumn=min(6,double(predictionStep)+1);
    state.iabcPrediction(:,currentColumn)=iabcNext;
end
candidateExhausted=state.candidatePosition(idx)>uint8(2);
memory=state;
end

== matlab function FCSMPC_double_vector_2025b/FCS_MPC/SDA_Solve/SDA Solve/PSPL_TestFrame/SDA_PL_Framework/MetricCompare ==
  data: level input uint8 size=[1 1]; currentMetric output double size=[1 1]; quadraticMetric input double size=[1 1]; vectorMetric input double size=[1 1]; vectorCmvMetric input double size=[1 1]; memory input Bus: SdaMemoryBus size=[1 1]; best input Bus: SdaBestBus size=[1 1]; currentCmvMetric output double size=[1 1]; better output boolean size=[1 1]; prune output boolean size=[1 1]
function [currentMetric,currentCmvMetric,better,prune] = MetricCompare(level,quadraticMetric,vectorMetric,vectorCmvMetric,memory,best)
%#codegen
idx=max(uint8(1),min(uint8(15),level));
if mod(idx,uint8(3))==uint8(0)
 currentMetric=vectorMetric; currentCmvMetric=vectorCmvMetric;
else
 currentMetric=quadraticMetric;
 currentCmvMetric=memory.cmvMetricStack(double(idx)+1);
end
better=currentMetric<best.bestMetric;
prune=currentMetric>best.bestMetric;
end

== matlab function FCSMPC_double_vector_2025b/FCS_MPC/SDA_Solve/SDA Solve/PSPL_TestFrame/SDA_PL_Framework/ProblemLatch ==
  data: problemIn input Bus: SdaProblemBus size=[1 1]; problem output Bus: SdaProblemBus size=[1 1]; loadEnable input boolean size=[1 1]
function problem = ProblemLatch(problemIn, loadEnable)
%#codegen
persistent latchedProblem
if isempty(latchedProblem)
    latchedProblem = problemIn;
end
if loadEnable
    latchedProblem = problemIn;
end
problem = latchedProblem;
